simulink model "ASM_Traffic_MultiCore"  (R2026a)
settings: Solver=ode1  StartTime=SIM.tstart.v  StopTime=SIM.tend.v  FixedStep=SIM.StepSize.v
PostLoadFcn:
  | if any(exist('dsrtsu_mdlpostloadfcn', 'file') ~= 0), dsrtsu_mdlpostloadfcn('Execute', bdroot); end
  | try, asm_mdl_postloadfcn(bdroot, 'UpdateModel', 3600); catch, disp(lasterr); end,
InitFcn:
  | , if any(exist('rtifpga_mdlclblib', 'file') ~= 0), rtifpga_mdlclblib('Init', bdroot); end,
  | , if any(exist('dsmpb_private', 'file') ~= 0), dsmpb_private('dsmpb_mdlclblib', 'Init', bdroot); end,
model workspace (MAT data in the model file):
  asmReferencePath = [0 0.01 0.02 0.03 0.04 0.05 0.06 0.07 0.08 0.09 0.1 0.11 ... (350007 elements, 50001x7)]
  roadBounds : Simulink.Parameter (value not decoded)
  safetyAxes : Simulink.Parameter (value not decoded)
undefined symbols (not defined in the file): _to_, a0b2, ASM_BrakeHydraulics_DemoSystems, ASM_VehicleDynamics_DemoSystems, b98103fe8ad365046cd0, BrakeCircuit, controllerConfig, CPT, Crankshaft, DiscIntNeverNeededParam, dsmsi, FinalDriveAssembly, MDL, ModeSignals, mu, Pos_BrakePedal_Maneuver, rad, RefSignals, roadFamilyData, roadFamilyId, s_to_rpm, SIM, SoftECU, Suspension, Tire, Transmission
libraries: ASM_Traffic_lib x135, simulink x98, ASM_Utils_lib x77, ASM_VehicleDynamics_lib x70, ASM_Environment_lib x22, dsmpblib x20, dsmsilib x15, MDLD_Utils_lib x10, ASM_BrakeHydraulics_lib x3, sl_discontinuities x2
(part 60 of 65)

== system ASM_Traffic_MultiCore/Environment/Sensors/UserInterface/DISP_Plant/Object_Sensor_2D/Object_Sensor_2D_VisualizationData/Sensor_1_Front_Long ==
  Sensor : Inport
  Angle_Hor_Rel[deg] : Gain
  Angle_ScopeZone_Horizontal[deg] : Gain
  Angle_z_Orientation_Sensor_CoorSys_V[deg] : Gain
  Bus Selector : BusSelector  OutputSignals=Parameters.Sensor_Enable[0Off|1On],Parameters.Sensor_Detection_Mode[1Ray|2Sector],Parameters.Length_ScopeZone[m],Parameters.Pos_Sensor_Apex_CoorSys_V[x;y;z][m],Parameters.Angle_z_Orientation_Sensor_CoorSys_V[deg],Parameters.Angle_ScopeZone_Horizontal[deg],Parameters.SensorIdx[],SensorOutput.Object_ID[],SensorOutput.Distance[m],SensorOutput.Angle_Hor_Rel[deg]
  Distance[m] : Gain
  Length_ScopeZone[m] : Gain
  Object_ID[] : Gain
  Pos_Sensor_Apex_CoorSys_V[x;y;z][m] : Gain
  SensorIdx[] : Gain
  Sensor_Detection_Mode[1Ray|2Sector] : Gain
  Sensor_Enable[0Off|1On] : Gain
  Terminator{,1..9} (10 alike) : Terminator
  wires:
  Sensor/1 -> Bus Selector/1
  Bus Selector/1 -> Sensor_Enable[0Off|1On]/1  "<Sensor_Enable[0Off|1On]>"
  Sensor_Enable[0Off|1On]/1 -> Terminator/1
  Sensor_Detection_Mode[1Ray|2Sector]/1 -> Terminator1/1
  Bus Selector/2 -> Sensor_Detection_Mode[1Ray|2Sector]/1  "<Sensor_Detection_Mode[1Ray|2Sector]>"
  Pos_Sensor_Apex_CoorSys_V[x;y;z][m]/1 -> Terminator2/1
  Angle_z_Orientation_Sensor_CoorSys_V[deg]/1 -> Terminator3/1
  Angle_ScopeZone_Horizontal[deg]/1 -> Terminator4/1
  SensorIdx[]/1 -> Terminator5/1
  Object_ID[]/1 -> Terminator6/1
  Distance[m]/1 -> Terminator7/1
  Angle_Hor_Rel[deg]/1 -> Terminator8/1
  Bus Selector/4 -> Pos_Sensor_Apex_CoorSys_V[x;y;z][m]/1  "<Pos_Sensor_Apex_CoorSys_V[x;y;z][m]>"
  Bus Selector/5 -> Angle_z_Orientation_Sensor_CoorSys_V[deg]/1  "<Angle_z_Orientation_Sensor_CoorSys_V[deg]>"
  Bus Selector/6 -> Angle_ScopeZone_Horizontal[deg]/1  "<Angle_ScopeZone_Horizontal[deg]>"
  Bus Selector/7 -> SensorIdx[]/1  "<SensorIdx[]>"
  Bus Selector/8 -> Object_ID[]/1  "<Object_ID[]>"
  Bus Selector/9 -> Distance[m]/1  "<Distance[m]>"
  Bus Selector/10 -> Angle_Hor_Rel[deg]/1  "<Angle_Hor_Rel[deg]>"
  Length_ScopeZone[m]/1 -> Terminator9/1
  Bus Selector/3 -> Length_ScopeZone[m]/1  "<Length_ScopeZone[m]>"

== system ASM_Traffic_MultiCore/Environment/Sensors/UserInterface/DISP_Plant/Object_Sensor_2D/Object_Sensor_2D_VisualizationData/Sensor_2_Front_Left ==
  Sensor : Inport
  Angle_Hor_Rel[deg] : Gain
  Angle_ScopeZone_Horizontal[deg] : Gain
  Angle_z_Orientation_Sensor_CoorSys_V[deg] : Gain
  Bus Selector : BusSelector  OutputSignals=Parameters.Sensor_Enable[0Off|1On],Parameters.Sensor_Detection_Mode[1Ray|2Sector],Parameters.Length_ScopeZone[m],Parameters.Pos_Sensor_Apex_CoorSys_V[x;y;z][m],Parameters.Angle_z_Orientation_Sensor_CoorSys_V[deg],Parameters.Angle_ScopeZone_Horizontal[deg],Parameters.SensorIdx[],SensorOutput.Object_ID[],SensorOutput.Distance[m],SensorOutput.Angle_Hor_Rel[deg]
  Distance[m] : Gain
  Length_ScopeZone[m] : Gain
  Object_ID[] : Gain
  Pos_Sensor_Apex_CoorSys_V[x;y;z][m] : Gain
  SensorIdx[] : Gain
  Sensor_Detection_Mode[1Ray|2Sector] : Gain
  Sensor_Enable[0Off|1On] : Gain
  Terminator{,1..9} (10 alike) : Terminator
  wires:
  Bus Selector/3 -> Length_ScopeZone[m]/1  "<Length_ScopeZone[m]>"
  Length_ScopeZone[m]/1 -> Terminator9/1
  Bus Selector/10 -> Angle_Hor_Rel[deg]/1  "<Angle_Hor_Rel[deg]>"
  Bus Selector/9 -> Distance[m]/1  "<Distance[m]>"
  Bus Selector/8 -> Object_ID[]/1  "<Object_ID[]>"
  Bus Selector/7 -> SensorIdx[]/1  "<SensorIdx[]>"
  Bus Selector/6 -> Angle_ScopeZone_Horizontal[deg]/1  "<Angle_ScopeZone_Horizontal[deg]>"
  Bus Selector/5 -> Angle_z_Orientation_Sensor_CoorSys_V[deg]/1  "<Angle_z_Orientation_Sensor_CoorSys_V[deg]>"
  Bus Selector/4 -> Pos_Sensor_Apex_CoorSys_V[x;y;z][m]/1  "<Pos_Sensor_Apex_CoorSys_V[x;y;z][m]>"
  Angle_Hor_Rel[deg]/1 -> Terminator8/1
  Distance[m]/1 -> Terminator7/1
  Object_ID[]/1 -> Terminator6/1
  SensorIdx[]/1 -> Terminator5/1
  Angle_ScopeZone_Horizontal[deg]/1 -> Terminator4/1
  Angle_z_Orientation_Sensor_CoorSys_V[deg]/1 -> Terminator3/1
  Pos_Sensor_Apex_CoorSys_V[x;y;z][m]/1 -> Terminator2/1
  Bus Selector/2 -> Sensor_Detection_Mode[1Ray|2Sector]/1  "<Sensor_Detection_Mode[1Ray|2Sector]>"
  Sensor_Detection_Mode[1Ray|2Sector]/1 -> Terminator1/1
  Sensor_Enable[0Off|1On]/1 -> Terminator/1
  Bus Selector/1 -> Sensor_Enable[0Off|1On]/1  "<Sensor_Enable[0Off|1On]>"
  Sensor/1 -> Bus Selector/1

== system ASM_Traffic_MultiCore/Environment/Sensors/UserInterface/DISP_Plant/Object_Sensor_2D/Object_Sensor_2D_VisualizationData/Sensor_3_Left ==
  Sensor : Inport
  Angle_Hor_Rel[deg] : Gain
  Angle_ScopeZone_Horizontal[deg] : Gain
  Angle_z_Orientation_Sensor_CoorSys_V[deg] : Gain
  Bus Selector : BusSelector  OutputSignals=Parameters.Sensor_Enable[0Off|1On],Parameters.Sensor_Detection_Mode[1Ray|2Sector],Parameters.Length_ScopeZone[m],Parameters.Pos_Sensor_Apex_CoorSys_V[x;y;z][m],Parameters.Angle_z_Orientation_Sensor_CoorSys_V[deg],Parameters.Angle_ScopeZone_Horizontal[deg],Parameters.SensorIdx[],SensorOutput.Object_ID[],SensorOutput.Distance[m],SensorOutput.Angle_Hor_Rel[deg]
  Distance[m] : Gain
  Length_ScopeZone[m] : Gain
  Object_ID[] : Gain
  Pos_Sensor_Apex_CoorSys_V[x;y;z][m] : Gain
  SensorIdx[] : Gain
  Sensor_Detection_Mode[1Ray|2Sector] : Gain
  Sensor_Enable[0Off|1On] : Gain
  Terminator{,1..9} (10 alike) : Terminator
  wires:
  Sensor/1 -> Bus Selector/1
  Bus Selector/1 -> Sensor_Enable[0Off|1On]/1  "<Sensor_Enable[0Off|1On]>"
  Sensor_Enable[0Off|1On]/1 -> Terminator/1
  Sensor_Detection_Mode[1Ray|2Sector]/1 -> Terminator1/1
  Bus Selector/2 -> Sensor_Detection_Mode[1Ray|2Sector]/1  "<Sensor_Detection_Mode[1Ray|2Sector]>"
  Pos_Sensor_Apex_CoorSys_V[x;y;z][m]/1 -> Terminator2/1
  Angle_z_Orientation_Sensor_CoorSys_V[deg]/1 -> Terminator3/1
  Angle_ScopeZone_Horizontal[deg]/1 -> Terminator4/1
  SensorIdx[]/1 -> Terminator5/1
  Object_ID[]/1 -> Terminator6/1
  Distance[m]/1 -> Terminator7/1
  Angle_Hor_Rel[deg]/1 -> Terminator8/1
  Bus Selector/4 -> Pos_Sensor_Apex_CoorSys_V[x;y;z][m]/1  "<Pos_Sensor_Apex_CoorSys_V[x;y;z][m]>"
  Bus Selector/5 -> Angle_z_Orientation_Sensor_CoorSys_V[deg]/1  "<Angle_z_Orientation_Sensor_CoorSys_V[deg]>"
  Bus Selector/6 -> Angle_ScopeZone_Horizontal[deg]/1  "<Angle_ScopeZone_Horizontal[deg]>"
  Bus Selector/7 -> SensorIdx[]/1  "<SensorIdx[]>"
  Bus Selector/8 -> Object_ID[]/1  "<Object_ID[]>"
  Bus Selector/9 -> Distance[m]/1  "<Distance[m]>"
  Bus Selector/10 -> Angle_Hor_Rel[deg]/1  "<Angle_Hor_Rel[deg]>"
  Length_ScopeZone[m]/1 -> Terminator9/1
  Bus Selector/3 -> Length_ScopeZone[m]/1  "<Length_ScopeZone[m]>"

== system ASM_Traffic_MultiCore/Environment/Sensors/UserInterface/DISP_Plant/Object_Sensor_2D/Object_Sensor_2D_VisualizationData/Sensor_4_Rear_Left ==
  Sensor : Inport
  Angle_Hor_Rel[deg] : Gain
  Angle_ScopeZone_Horizontal[deg] : Gain
  Angle_z_Orientation_Sensor_CoorSys_V[deg] : Gain
  Bus Selector : BusSelector  OutputSignals=Parameters.Sensor_Enable[0Off|1On],Parameters.Sensor_Detection_Mode[1Ray|2Sector],Parameters.Length_ScopeZone[m],Parameters.Pos_Sensor_Apex_CoorSys_V[x;y;z][m],Parameters.Angle_z_Orientation_Sensor_CoorSys_V[deg],Parameters.Angle_ScopeZone_Horizontal[deg],Parameters.SensorIdx[],SensorOutput.Object_ID[],SensorOutput.Distance[m],SensorOutput.Angle_Hor_Rel[deg]
  Distance[m] : Gain
  Length_ScopeZone[m] : Gain
  Object_ID[] : Gain
  Pos_Sensor_Apex_CoorSys_V[x;y;z][m] : Gain
  SensorIdx[] : Gain
  Sensor_Detection_Mode[1Ray|2Sector] : Gain
  Sensor_Enable[0Off|1On] : Gain
  Terminator{,1..9} (10 alike) : Terminator
  wires:
  Bus Selector/3 -> Length_ScopeZone[m]/1  "<Length_ScopeZone[m]>"
  Length_ScopeZone[m]/1 -> Terminator9/1
  Bus Selector/10 -> Angle_Hor_Rel[deg]/1  "<Angle_Hor_Rel[deg]>"
  Bus Selector/9 -> Distance[m]/1  "<Distance[m]>"
  Bus Selector/8 -> Object_ID[]/1  "<Object_ID[]>"
  Bus Selector/7 -> SensorIdx[]/1  "<SensorIdx[]>"
  Bus Selector/6 -> Angle_ScopeZone_Horizontal[deg]/1  "<Angle_ScopeZone_Horizontal[deg]>"
  Bus Selector/5 -> Angle_z_Orientation_Sensor_CoorSys_V[deg]/1  "<Angle_z_Orientation_Sensor_CoorSys_V[deg]>"
  Bus Selector/4 -> Pos_Sensor_Apex_CoorSys_V[x;y;z][m]/1  "<Pos_Sensor_Apex_CoorSys_V[x;y;z][m]>"
  Angle_Hor_Rel[deg]/1 -> Terminator8/1
  Distance[m]/1 -> Terminator7/1
  Object_ID[]/1 -> Terminator6/1
  SensorIdx[]/1 -> Terminator5/1
  Angle_ScopeZone_Horizontal[deg]/1 -> Terminator4/1
  Angle_z_Orientation_Sensor_CoorSys_V[deg]/1 -> Terminator3/1
  Pos_Sensor_Apex_CoorSys_V[x;y;z][m]/1 -> Terminator2/1
  Bus Selector/2 -> Sensor_Detection_Mode[1Ray|2Sector]/1  "<Sensor_Detection_Mode[1Ray|2Sector]>"
  Sensor_Detection_Mode[1Ray|2Sector]/1 -> Terminator1/1
  Sensor_Enable[0Off|1On]/1 -> Terminator/1
  Bus Selector/1 -> Sensor_Enable[0Off|1On]/1  "<Sensor_Enable[0Off|1On]>"
  Sensor/1 -> Bus Selector/1

== system ASM_Traffic_MultiCore/Environment/Sensors/UserInterface/DISP_Plant/Object_Sensor_2D/Object_Sensor_2D_VisualizationData/Sensor_5_Front_Right ==
  Sensor : Inport
  Angle_Hor_Rel[deg] : Gain
  Angle_ScopeZone_Horizontal[deg] : Gain
  Angle_z_Orientation_Sensor_CoorSys_V[deg] : Gain
  Bus Selector : BusSelector  OutputSignals=Parameters.Sensor_Enable[0Off|1On],Parameters.Sensor_Detection_Mode[1Ray|2Sector],Parameters.Length_ScopeZone[m],Parameters.Pos_Sensor_Apex_CoorSys_V[x;y;z][m],Parameters.Angle_z_Orientation_Sensor_CoorSys_V[deg],Parameters.Angle_ScopeZone_Horizontal[deg],Parameters.SensorIdx[],SensorOutput.Object_ID[],SensorOutput.Distance[m],SensorOutput.Angle_Hor_Rel[deg]
  Distance[m] : Gain
  Length_ScopeZone[m] : Gain
  Object_ID[] : Gain
  Pos_Sensor_Apex_CoorSys_V[x;y;z][m] : Gain
  SensorIdx[] : Gain
  Sensor_Detection_Mode[1Ray|2Sector] : Gain
  Sensor_Enable[0Off|1On] : Gain
  Terminator{,1..9} (10 alike) : Terminator
  wires:
  Sensor/1 -> Bus Selector/1
  Bus Selector/1 -> Sensor_Enable[0Off|1On]/1  "<Sensor_Enable[0Off|1On]>"
  Sensor_Enable[0Off|1On]/1 -> Terminator/1
  Sensor_Detection_Mode[1Ray|2Sector]/1 -> Terminator1/1
  Bus Selector/2 -> Sensor_Detection_Mode[1Ray|2Sector]/1  "<Sensor_Detection_Mode[1Ray|2Sector]>"
  Pos_Sensor_Apex_CoorSys_V[x;y;z][m]/1 -> Terminator2/1
  Angle_z_Orientation_Sensor_CoorSys_V[deg]/1 -> Terminator3/1
  Angle_ScopeZone_Horizontal[deg]/1 -> Terminator4/1
  SensorIdx[]/1 -> Terminator5/1
  Object_ID[]/1 -> Terminator6/1
  Distance[m]/1 -> Terminator7/1
  Angle_Hor_Rel[deg]/1 -> Terminator8/1
  Bus Selector/4 -> Pos_Sensor_Apex_CoorSys_V[x;y;z][m]/1  "<Pos_Sensor_Apex_CoorSys_V[x;y;z][m]>"
  Bus Selector/5 -> Angle_z_Orientation_Sensor_CoorSys_V[deg]/1  "<Angle_z_Orientation_Sensor_CoorSys_V[deg]>"
  Bus Selector/6 -> Angle_ScopeZone_Horizontal[deg]/1  "<Angle_ScopeZone_Horizontal[deg]>"
  Bus Selector/7 -> SensorIdx[]/1  "<SensorIdx[]>"
  Bus Selector/8 -> Object_ID[]/1  "<Object_ID[]>"
  Bus Selector/9 -> Distance[m]/1  "<Distance[m]>"
  Bus Selector/10 -> Angle_Hor_Rel[deg]/1  "<Angle_Hor_Rel[deg]>"
  Length_ScopeZone[m]/1 -> Terminator9/1
  Bus Selector/3 -> Length_ScopeZone[m]/1  "<Length_ScopeZone[m]>"

== system ASM_Traffic_MultiCore/Environment/Sensors/UserInterface/DISP_Plant/Object_Sensor_2D/Object_Sensor_2D_VisualizationData/Sensor_6_Right ==
  Sensor : Inport
  Angle_Hor_Rel[deg] : Gain
  Angle_ScopeZone_Horizontal[deg] : Gain
  Angle_z_Orientation_Sensor_CoorSys_V[deg] : Gain
  Bus Selector : BusSelector  OutputSignals=Parameters.Sensor_Enable[0Off|1On],Parameters.Sensor_Detection_Mode[1Ray|2Sector],Parameters.Length_ScopeZone[m],Parameters.Pos_Sensor_Apex_CoorSys_V[x;y;z][m],Parameters.Angle_z_Orientation_Sensor_CoorSys_V[deg],Parameters.Angle_ScopeZone_Horizontal[deg],Parameters.SensorIdx[],SensorOutput.Object_ID[],SensorOutput.Distance[m],SensorOutput.Angle_Hor_Rel[deg]
  Distance[m] : Gain
  Length_ScopeZone[m] : Gain
  Object_ID[] : Gain
  Pos_Sensor_Apex_CoorSys_V[x;y;z][m] : Gain
  SensorIdx[] : Gain
  Sensor_Detection_Mode[1Ray|2Sector] : Gain
  Sensor_Enable[0Off|1On] : Gain
  Terminator{,1..9} (10 alike) : Terminator
  wires:
  Bus Selector/3 -> Length_ScopeZone[m]/1  "<Length_ScopeZone[m]>"
  Length_ScopeZone[m]/1 -> Terminator9/1
  Bus Selector/10 -> Angle_Hor_Rel[deg]/1  "<Angle_Hor_Rel[deg]>"
  Bus Selector/9 -> Distance[m]/1  "<Distance[m]>"
  Bus Selector/8 -> Object_ID[]/1  "<Object_ID[]>"
  Bus Selector/7 -> SensorIdx[]/1  "<SensorIdx[]>"
  Bus Selector/6 -> Angle_ScopeZone_Horizontal[deg]/1  "<Angle_ScopeZone_Horizontal[deg]>"
  Bus Selector/5 -> Angle_z_Orientation_Sensor_CoorSys_V[deg]/1  "<Angle_z_Orientation_Sensor_CoorSys_V[deg]>"
  Bus Selector/4 -> Pos_Sensor_Apex_CoorSys_V[x;y;z][m]/1  "<Pos_Sensor_Apex_CoorSys_V[x;y;z][m]>"
  Angle_Hor_Rel[deg]/1 -> Terminator8/1
  Distance[m]/1 -> Terminator7/1
  Object_ID[]/1 -> Terminator6/1
  SensorIdx[]/1 -> Terminator5/1
  Angle_ScopeZone_Horizontal[deg]/1 -> Terminator4/1
  Angle_z_Orientation_Sensor_CoorSys_V[deg]/1 -> Terminator3/1
  Pos_Sensor_Apex_CoorSys_V[x;y;z][m]/1 -> Terminator2/1
  Bus Selector/2 -> Sensor_Detection_Mode[1Ray|2Sector]/1  "<Sensor_Detection_Mode[1Ray|2Sector]>"
  Sensor_Detection_Mode[1Ray|2Sector]/1 -> Terminator1/1
  Sensor_Enable[0Off|1On]/1 -> Terminator/1
  Bus Selector/1 -> Sensor_Enable[0Off|1On]/1  "<Sensor_Enable[0Off|1On]>"
  Sensor/1 -> Bus Selector/1

== system ASM_Traffic_MultiCore/Environment/Sensors/UserInterface/DISP_Plant/Object_Sensor_2D/Object_Sensor_2D_VisualizationData/Sensor_7_Rear_Right ==
  Sensor : Inport
  Angle_Hor_Rel[deg] : Gain
  Angle_ScopeZone_Horizontal[deg] : Gain
  Angle_z_Orientation_Sensor_CoorSys_V[deg] : Gain
  Bus Selector : BusSelector  OutputSignals=Parameters.Sensor_Enable[0Off|1On],Parameters.Sensor_Detection_Mode[1Ray|2Sector],Parameters.Length_ScopeZone[m],Parameters.Pos_Sensor_Apex_CoorSys_V[x;y;z][m],Parameters.Angle_z_Orientation_Sensor_CoorSys_V[deg],Parameters.Angle_ScopeZone_Horizontal[deg],Parameters.SensorIdx[],SensorOutput.Object_ID[],SensorOutput.Distance[m],SensorOutput.Angle_Hor_Rel[deg]
  Distance[m] : Gain
  Length_ScopeZone[m] : Gain
  Object_ID[] : Gain
  Pos_Sensor_Apex_CoorSys_V[x;y;z][m] : Gain
  SensorIdx[] : Gain
  Sensor_Detection_Mode[1Ray|2Sector] : Gain
  Sensor_Enable[0Off|1On] : Gain
  Terminator{,1..9} (10 alike) : Terminator
  wires:
  Sensor/1 -> Bus Selector/1
  Bus Selector/1 -> Sensor_Enable[0Off|1On]/1  "<Sensor_Enable[0Off|1On]>"
  Sensor_Enable[0Off|1On]/1 -> Terminator/1
  Sensor_Detection_Mode[1Ray|2Sector]/1 -> Terminator1/1
  Bus Selector/2 -> Sensor_Detection_Mode[1Ray|2Sector]/1  "<Sensor_Detection_Mode[1Ray|2Sector]>"
  Pos_Sensor_Apex_CoorSys_V[x;y;z][m]/1 -> Terminator2/1
  Angle_z_Orientation_Sensor_CoorSys_V[deg]/1 -> Terminator3/1
  Angle_ScopeZone_Horizontal[deg]/1 -> Terminator4/1
  SensorIdx[]/1 -> Terminator5/1
  Object_ID[]/1 -> Terminator6/1
  Distance[m]/1 -> Terminator7/1
  Angle_Hor_Rel[deg]/1 -> Terminator8/1
  Bus Selector/4 -> Pos_Sensor_Apex_CoorSys_V[x;y;z][m]/1  "<Pos_Sensor_Apex_CoorSys_V[x;y;z][m]>"
  Bus Selector/5 -> Angle_z_Orientation_Sensor_CoorSys_V[deg]/1  "<Angle_z_Orientation_Sensor_CoorSys_V[deg]>"
  Bus Selector/6 -> Angle_ScopeZone_Horizontal[deg]/1  "<Angle_ScopeZone_Horizontal[deg]>"
  Bus Selector/7 -> SensorIdx[]/1  "<SensorIdx[]>"
  Bus Selector/8 -> Object_ID[]/1  "<Object_ID[]>"
  Bus Selector/9 -> Distance[m]/1  "<Distance[m]>"
  Bus Selector/10 -> Angle_Hor_Rel[deg]/1  "<Angle_Hor_Rel[deg]>"
  Length_ScopeZone[m]/1 -> Terminator9/1
  Bus Selector/3 -> Length_ScopeZone[m]/1  "<Length_ScopeZone[m]>"

== system ASM_Traffic_MultiCore/Environment/Sensors/UserInterface/DISP_Plant/Object_Sensor_3D/IdxSelect_3DSensor/Angle_Hor_Object_1[deg] ==
  In1 : Inport
  Out1 : Outport  VectorParamsAs1DForOutWhenUnconnected=off
  wires:
  In1/1 -> Out1/1

== system ASM_Traffic_MultiCore/Environment/Sensors/UserInterface/DISP_Plant/Object_Sensor_3D/IdxSelect_3DSensor/Angle_Hor_Object_2[deg] ==
  In1 : Inport
  Out1 : Outport  VectorParamsAs1DForOutWhenUnconnected=off
  wires:
  In1/1 -> Out1/1

== system ASM_Traffic_MultiCore/Environment/Sensors/UserInterface/DISP_Plant/Object_Sensor_3D/IdxSelect_3DSensor/Angle_Hor_Object_3[deg] ==
  In1 : Inport
  Out1 : Outport  VectorParamsAs1DForOutWhenUnconnected=off
  wires:
  In1/1 -> Out1/1

== system ASM_Traffic_MultiCore/Environment/Sensors/UserInterface/DISP_Plant/Object_Sensor_3D/IdxSelect_3DSensor/Angle_Ver_Object_1[deg] ==
  In1 : Inport
  Out1 : Outport  VectorParamsAs1DForOutWhenUnconnected=off
  wires:
  In1/1 -> Out1/1

== system ASM_Traffic_MultiCore/Environment/Sensors/UserInterface/DISP_Plant/Object_Sensor_3D/IdxSelect_3DSensor/Angle_Ver_Object_2[deg] ==
  In1 : Inport
  Out1 : Outport  VectorParamsAs1DForOutWhenUnconnected=off
  wires:
  In1/1 -> Out1/1

== system ASM_Traffic_MultiCore/Environment/Sensors/UserInterface/DISP_Plant/Object_Sensor_3D/IdxSelect_3DSensor/Angle_Ver_Object_3[deg] ==
  In1 : Inport
  Out1 : Outport  VectorParamsAs1DForOutWhenUnconnected=off
  wires:
  In1/1 -> Out1/1

== system ASM_Traffic_MultiCore/Environment/Sensors/UserInterface/DISP_Plant/Object_Sensor_3D/IdxSelect_3DSensor/Angle_x_Objects_CoorSysE_1[deg] ==
  In1 : Inport
  Out1 : Outport  VectorParamsAs1DForOutWhenUnconnected=off
  wires:
  In1/1 -> Out1/1

== system ASM_Traffic_MultiCore/Environment/Sensors/UserInterface/DISP_Plant/Object_Sensor_3D/IdxSelect_3DSensor/Angle_x_Objects_CoorSysE_2[deg] ==
  In1 : Inport
  Out1 : Outport  VectorParamsAs1DForOutWhenUnconnected=off
  wires:
  In1/1 -> Out1/1

== system ASM_Traffic_MultiCore/Environment/Sensors/UserInterface/DISP_Plant/Object_Sensor_3D/IdxSelect_3DSensor/Angle_x_Objects_CoorSysE_3[deg] ==
  In1 : Inport
  Out1 : Outport  VectorParamsAs1DForOutWhenUnconnected=off
  wires:
  In1/1 -> Out1/1

== system ASM_Traffic_MultiCore/Environment/Sensors/UserInterface/DISP_Plant/Object_Sensor_3D/IdxSelect_3DSensor/Angle_y_Objects_CoorSysE_1[deg] ==
  In1 : Inport
  Out1 : Outport  VectorParamsAs1DForOutWhenUnconnected=off
  wires:
  In1/1 -> Out1/1

== system ASM_Traffic_MultiCore/Environment/Sensors/UserInterface/DISP_Plant/Object_Sensor_3D/IdxSelect_3DSensor/Angle_y_Objects_CoorSysE_2[deg] ==
  In1 : Inport
  Out1 : Outport  VectorParamsAs1DForOutWhenUnconnected=off
  wires:
  In1/1 -> Out1/1

== system ASM_Traffic_MultiCore/Environment/Sensors/UserInterface/DISP_Plant/Object_Sensor_3D/IdxSelect_3DSensor/Angle_y_Objects_CoorSysE_3[deg] ==
  In1 : Inport
  Out1 : Outport  VectorParamsAs1DForOutWhenUnconnected=off
  wires:
  In1/1 -> Out1/1

== system ASM_Traffic_MultiCore/Environment/Sensors/UserInterface/DISP_Plant/Object_Sensor_3D/IdxSelect_3DSensor/Angle_z_Objects_CoorSysE_1[deg] ==
  In1 : Inport
  Out1 : Outport  VectorParamsAs1DForOutWhenUnconnected=off
  wires:
  In1/1 -> Out1/1

== system ASM_Traffic_MultiCore/Environment/Sensors/UserInterface/DISP_Plant/Object_Sensor_3D/IdxSelect_3DSensor/Angle_z_Objects_CoorSysE_2[deg] ==
  In1 : Inport
  Out1 : Outport  VectorParamsAs1DForOutWhenUnconnected=off
  wires:
  In1/1 -> Out1/1

== system ASM_Traffic_MultiCore/Environment/Sensors/UserInterface/DISP_Plant/Object_Sensor_3D/IdxSelect_3DSensor/Angle_z_Objects_CoorSysE_3[deg] ==
  In1 : Inport
  Out1 : Outport  VectorParamsAs1DForOutWhenUnconnected=off
  wires:
  In1/1 -> Out1/1

== system ASM_Traffic_MultiCore/Environment/Sensors/UserInterface/DISP_Plant/Object_Sensor_3D/IdxSelect_3DSensor/CustomPoint_Angle_Hor_CoorSys_S_1[deg] ==
  In1 : Inport
  Out1 : Outport  VectorParamsAs1DForOutWhenUnconnected=off
  wires:
  In1/1 -> Out1/1

== system ASM_Traffic_MultiCore/Environment/Sensors/UserInterface/DISP_Plant/Object_Sensor_3D/IdxSelect_3DSensor/CustomPoint_Angle_Hor_CoorSys_S_2[deg] ==
  In1 : Inport
  Out1 : Outport  VectorParamsAs1DForOutWhenUnconnected=off
  wires:
  In1/1 -> Out1/1

== system ASM_Traffic_MultiCore/Environment/Sensors/UserInterface/DISP_Plant/Object_Sensor_3D/IdxSelect_3DSensor/CustomPoint_Angle_Hor_CoorSys_S_3[deg] ==
  In1 : Inport
  Out1 : Outport  VectorParamsAs1DForOutWhenUnconnected=off
  wires:
  In1/1 -> Out1/1

== system ASM_Traffic_MultiCore/Environment/Sensors/UserInterface/DISP_Plant/Object_Sensor_3D/IdxSelect_3DSensor/CustomPoint_Dist_CoorSys_S_1[m] ==
  In1 : Inport
  Out1 : Outport  VectorParamsAs1DForOutWhenUnconnected=off
  wires:
  In1/1 -> Out1/1

== system ASM_Traffic_MultiCore/Environment/Sensors/UserInterface/DISP_Plant/Object_Sensor_3D/IdxSelect_3DSensor/CustomPoint_Dist_CoorSys_S_2[m] ==
  In1 : Inport
  Out1 : Outport  VectorParamsAs1DForOutWhenUnconnected=off
  wires:
  In1/1 -> Out1/1

== system ASM_Traffic_MultiCore/Environment/Sensors/UserInterface/DISP_Plant/Object_Sensor_3D/IdxSelect_3DSensor/CustomPoint_Dist_CoorSys_S_3[m] ==
  In1 : Inport
  Out1 : Outport  VectorParamsAs1DForOutWhenUnconnected=off
  wires:
  In1/1 -> Out1/1

== system ASM_Traffic_MultiCore/Environment/Sensors/UserInterface/DISP_Plant/Object_Sensor_3D/IdxSelect_3DSensor/CustomPoint_ID_1[] ==
  In1 : Inport
  Out1 : Outport  VectorParamsAs1DForOutWhenUnconnected=off
  wires:
  In1/1 -> Out1/1

== system ASM_Traffic_MultiCore/Environment/Sensors/UserInterface/DISP_Plant/Object_Sensor_3D/IdxSelect_3DSensor/CustomPoint_ID_2[] ==
  In1 : Inport
  Out1 : Outport  VectorParamsAs1DForOutWhenUnconnected=off
  wires:
  In1/1 -> Out1/1

== system ASM_Traffic_MultiCore/Environment/Sensors/UserInterface/DISP_Plant/Object_Sensor_3D/IdxSelect_3DSensor/CustomPoint_ID_3[] ==
  In1 : Inport
  Out1 : Outport  VectorParamsAs1DForOutWhenUnconnected=off
  wires:
  In1/1 -> Out1/1

== system ASM_Traffic_MultiCore/Environment/Sensors/UserInterface/DISP_Plant/Object_Sensor_3D/IdxSelect_3DSensor/CustomPoint_Pos_ObjectPoint_CoorSys_E_1[x;y;z][m] ==
  In1 : Inport
  Out1 : Outport  VectorParamsAs1DForOutWhenUnconnected=off
  wires:
  In1/1 -> Out1/1

== system ASM_Traffic_MultiCore/Environment/Sensors/UserInterface/DISP_Plant/Object_Sensor_3D/IdxSelect_3DSensor/CustomPoint_Pos_ObjectPoint_CoorSys_E_2[x;y;z][m] ==
  In1 : Inport
  Out1 : Outport  VectorParamsAs1DForOutWhenUnconnected=off
  wires:
  In1/1 -> Out1/1

== system ASM_Traffic_MultiCore/Environment/Sensors/UserInterface/DISP_Plant/Object_Sensor_3D/IdxSelect_3DSensor/CustomPoint_Pos_ObjectPoint_CoorSys_E_3[x;y;z][m] ==
  In1 : Inport
  Out1 : Outport  VectorParamsAs1DForOutWhenUnconnected=off
  wires:
  In1/1 -> Out1/1

== system ASM_Traffic_MultiCore/Environment/Sensors/UserInterface/DISP_Plant/Object_Sensor_3D/IdxSelect_3DSensor/CustomValues_1[] ==
  In1 : Inport
  Out1 : Outport  VectorParamsAs1DForOutWhenUnconnected=off
  wires:
  In1/1 -> Out1/1

== system ASM_Traffic_MultiCore/Environment/Sensors/UserInterface/DISP_Plant/Object_Sensor_3D/IdxSelect_3DSensor/CustomValues_2[] ==
  In1 : Inport
  Out1 : Outport  VectorParamsAs1DForOutWhenUnconnected=off
  wires:
  In1/1 -> Out1/1

== system ASM_Traffic_MultiCore/Environment/Sensors/UserInterface/DISP_Plant/Object_Sensor_3D/IdxSelect_3DSensor/CustomValues_3[] ==
  In1 : Inport
  Out1 : Outport  VectorParamsAs1DForOutWhenUnconnected=off
  wires:
  In1/1 -> Out1/1

== system ASM_Traffic_MultiCore/Environment/Sensors/UserInterface/DISP_Plant/Object_Sensor_3D/IdxSelect_3DSensor/Dist_Object_1[m] ==
  In1 : Inport
  Out1 : Outport  VectorParamsAs1DForOutWhenUnconnected=off
  wires:
  In1/1 -> Out1/1

== system ASM_Traffic_MultiCore/Environment/Sensors/UserInterface/DISP_Plant/Object_Sensor_3D/IdxSelect_3DSensor/Dist_Object_2[m] ==
  In1 : Inport
  Out1 : Outport  VectorParamsAs1DForOutWhenUnconnected=off
  wires:
  In1/1 -> Out1/1

== system ASM_Traffic_MultiCore/Environment/Sensors/UserInterface/DISP_Plant/Object_Sensor_3D/IdxSelect_3DSensor/Dist_Object_3[m] ==
  In1 : Inport
  Out1 : Outport  VectorParamsAs1DForOutWhenUnconnected=off
  wires:
  In1/1 -> Out1/1

== system ASM_Traffic_MultiCore/Environment/Sensors/UserInterface/DISP_Plant/Object_Sensor_3D/IdxSelect_3DSensor/Flag_BoxProperties_1[0|1] ==
  In1 : Inport
  Out1 : Outport  VectorParamsAs1DForOutWhenUnconnected=off
  wires:
  In1/1 -> Out1/1

== system ASM_Traffic_MultiCore/Environment/Sensors/UserInterface/DISP_Plant/Object_Sensor_3D/IdxSelect_3DSensor/Flag_BoxProperties_2[0|1] ==
  In1 : Inport
  Out1 : Outport  VectorParamsAs1DForOutWhenUnconnected=off
  wires:
  In1/1 -> Out1/1

== system ASM_Traffic_MultiCore/Environment/Sensors/UserInterface/DISP_Plant/Object_Sensor_3D/IdxSelect_3DSensor/Flag_BoxProperties_3[0|1] ==
  In1 : Inport
  Out1 : Outport  VectorParamsAs1DForOutWhenUnconnected=off
  wires:
  In1/1 -> Out1/1

== system ASM_Traffic_MultiCore/Environment/Sensors/UserInterface/DISP_Plant/Object_Sensor_3D/IdxSelect_3DSensor/Flag_NearestPnt_Occluded1[-1|0|1] ==
  In1 : Inport
  Out1 : Outport  VectorParamsAs1DForOutWhenUnconnected=off
  wires:
  In1/1 -> Out1/1

== system ASM_Traffic_MultiCore/Environment/Sensors/UserInterface/DISP_Plant/Object_Sensor_3D/IdxSelect_3DSensor/Flag_NearestPnt_Occluded2[-1|0|1] ==
  In1 : Inport
  Out1 : Outport  VectorParamsAs1DForOutWhenUnconnected=off
  wires:
  In1/1 -> Out1/1

== system ASM_Traffic_MultiCore/Environment/Sensors/UserInterface/DISP_Plant/Object_Sensor_3D/IdxSelect_3DSensor/Flag_NearestPnt_Occluded3[-1|0|1] ==
  In1 : Inport
  Out1 : Outport  VectorParamsAs1DForOutWhenUnconnected=off
  wires:
  In1/1 -> Out1/1

== system ASM_Traffic_MultiCore/Environment/Sensors/UserInterface/DISP_Plant/Object_Sensor_3D/IdxSelect_3DSensor/Flag_Object_In_Scope_1[0Out|1In] ==
  In1 : Inport
  Out1 : Outport  VectorParamsAs1DForOutWhenUnconnected=off
  wires:
  In1/1 -> Out1/1

== system ASM_Traffic_MultiCore/Environment/Sensors/UserInterface/DISP_Plant/Object_Sensor_3D/IdxSelect_3DSensor/Flag_Object_In_Scope_2[0Out|1In] ==
  In1 : Inport
  Out1 : Outport  VectorParamsAs1DForOutWhenUnconnected=off
  wires:
  In1/1 -> Out1/1

== system ASM_Traffic_MultiCore/Environment/Sensors/UserInterface/DISP_Plant/Object_Sensor_3D/IdxSelect_3DSensor/Flag_Object_In_Scope_3[0Out|1In] ==
  In1 : Inport
  Out1 : Outport  VectorParamsAs1DForOutWhenUnconnected=off
  wires:
  In1/1 -> Out1/1

== system ASM_Traffic_MultiCore/Environment/Sensors/UserInterface/DISP_Plant/Object_Sensor_3D/IdxSelect_3DSensor/Flag_Sensor_Apex_In_Object_1[0Out|1In] ==
  In1 : Inport
  Out1 : Outport  VectorParamsAs1DForOutWhenUnconnected=off
  wires:
  In1/1 -> Out1/1

== system ASM_Traffic_MultiCore/Environment/Sensors/UserInterface/DISP_Plant/Object_Sensor_3D/IdxSelect_3DSensor/Flag_Sensor_Apex_In_Object_2[0Out|1In] ==
  In1 : Inport
  Out1 : Outport  VectorParamsAs1DForOutWhenUnconnected=off
  wires:
  In1/1 -> Out1/1

== system ASM_Traffic_MultiCore/Environment/Sensors/UserInterface/DISP_Plant/Object_Sensor_3D/IdxSelect_3DSensor/Flag_Sensor_Apex_In_Object_3[0Out|1In] ==
  In1 : Inport
  Out1 : Outport  VectorParamsAs1DForOutWhenUnconnected=off
  wires:
  In1/1 -> Out1/1

== system ASM_Traffic_MultiCore/Environment/Sensors/UserInterface/DISP_Plant/Object_Sensor_3D/IdxSelect_3DSensor/Height_Object_1[m] ==
  In1 : Inport
  Out1 : Outport  VectorParamsAs1DForOutWhenUnconnected=off
  wires:
  In1/1 -> Out1/1

== system ASM_Traffic_MultiCore/Environment/Sensors/UserInterface/DISP_Plant/Object_Sensor_3D/IdxSelect_3DSensor/Height_Object_2[m] ==
  In1 : Inport
  Out1 : Outport  VectorParamsAs1DForOutWhenUnconnected=off
  wires:
  In1/1 -> Out1/1

== system ASM_Traffic_MultiCore/Environment/Sensors/UserInterface/DISP_Plant/Object_Sensor_3D/IdxSelect_3DSensor/Height_Object_3[m] ==
  In1 : Inport
  Out1 : Outport  VectorParamsAs1DForOutWhenUnconnected=off
  wires:
  In1/1 -> Out1/1

== system ASM_Traffic_MultiCore/Environment/Sensors/UserInterface/DISP_Plant/Object_Sensor_3D/IdxSelect_3DSensor/Length_Object_1[m] ==
  In1 : Inport
  Out1 : Outport  VectorParamsAs1DForOutWhenUnconnected=off
  wires:
  In1/1 -> Out1/1

== system ASM_Traffic_MultiCore/Environment/Sensors/UserInterface/DISP_Plant/Object_Sensor_3D/IdxSelect_3DSensor/Length_Object_2[m] ==
  In1 : Inport
  Out1 : Outport  VectorParamsAs1DForOutWhenUnconnected=off
  wires:
  In1/1 -> Out1/1

== system ASM_Traffic_MultiCore/Environment/Sensors/UserInterface/DISP_Plant/Object_Sensor_3D/IdxSelect_3DSensor/Length_Object_3[m] ==
  In1 : Inport
  Out1 : Outport  VectorParamsAs1DForOutWhenUnconnected=off
  wires:
  In1/1 -> Out1/1

== system ASM_Traffic_MultiCore/Environment/Sensors/UserInterface/DISP_Plant/Object_Sensor_3D/IdxSelect_3DSensor/MaskObjectData_CustomPoints_1 ==
  Object_ID_Expected[] : Inport
  Object_ID[] : Inport  Port=2
  ID[] : Inport  Port=3
  Dist_CoorSys_S[m] : Inport  Port=4
  Angle_Hor_CoorSys_S[deg] : Inport  Port=5
  Pos_ObjectPoint_CoorSys_E[x;y;z][m] : Inport  Port=6
  Demux : Demux  Outputs=3
  Mux : Mux  Inputs=3
  Product{,1..6} (7 alike) : Product
  Relational Operator1 : RelationalOperator  Operator===  OutDataTypeStr=boolean  RndMeth=Simplest  InputSameDT=off
  Object_ID_Masked[] : Outport
  ID_Masked[] : Outport  Port=2
  Dist_CoorSys_S_Masked[m] : Outport  Port=3
  Angle_Hor_CoorSys_S_Masked[deg] : Outport  Port=4
  Pos_ObjectPoint_CoorSys_E_Masked[x;y;z][m] : Outport  Port=5
  wires:
  Product6/1 -> Object_ID_Masked[]/1
  Demux/1 -> Product2/2
  Product5/1 -> Mux/3
  Product4/1 -> Mux/2
  Demux/2 -> Product4/2
  Relational Operator1/1 -> Product3/1, Product2/1, Product4/1, Product5/1, Product1/1, Product/1, Product6/1
  Product2/1 -> Mux/1
  Pos_ObjectPoint_CoorSys_E[x;y;z][m]/1 -> Demux/1
  Demux/3 -> Product5/2
  Object_ID[]/1 -> Relational Operator1/2, Product6/2
  Product1/1 -> Dist_CoorSys_S_Masked[m]/1
  Product3/1 -> Angle_Hor_CoorSys_S_Masked[deg]/1
  ID[]/1 -> Product/2
  Object_ID_Expected[]/1 -> Relational Operator1/1
  Product/1 -> ID_Masked[]/1
  Mux/1 -> Pos_ObjectPoint_CoorSys_E_Masked[x;y;z][m]/1
  Angle_Hor_CoorSys_S[deg]/1 -> Product3/2
  Dist_CoorSys_S[m]/1 -> Product1/2

== system ASM_Traffic_MultiCore/Environment/Sensors/UserInterface/DISP_Plant/Object_Sensor_3D/IdxSelect_3DSensor/MaskObjectData_CustomPoints_2 ==
  Object_ID_Expected[] : Inport
  Object_ID[] : Inport  Port=2
  ID[] : Inport  Port=3
  Dist_CoorSys_S[m] : Inport  Port=4
  Angle_Hor_CoorSys_S[deg] : Inport  Port=5
  Pos_ObjectPoint_CoorSys_E[x;y;z][m] : Inport  Port=6
  Demux : Demux  Outputs=3
  Mux : Mux  Inputs=3
  Product{,1..6} (7 alike) : Product
  Relational Operator1 : RelationalOperator  Operator===  OutDataTypeStr=boolean  RndMeth=Simplest  InputSameDT=off
  Object_ID_Masked[] : Outport
  ID_Masked[] : Outport  Port=2
  Dist_CoorSys_S_Masked[m] : Outport  Port=3
  Angle_Hor_CoorSys_S_Masked[deg] : Outport  Port=4
  Pos_ObjectPoint_CoorSys_E_Masked[x;y;z][m] : Outport  Port=5
  wires:
  Product6/1 -> Object_ID_Masked[]/1
  Demux/1 -> Product2/2
  Product5/1 -> Mux/3
  Product4/1 -> Mux/2
  Demux/2 -> Product4/2
  Relational Operator1/1 -> Product3/1, Product2/1, Product4/1, Product5/1, Product1/1, Product/1, Product6/1
  Product2/1 -> Mux/1
  Pos_ObjectPoint_CoorSys_E[x;y;z][m]/1 -> Demux/1
  Demux/3 -> Product5/2
  Object_ID[]/1 -> Relational Operator1/2, Product6/2
  Product1/1 -> Dist_CoorSys_S_Masked[m]/1
  Product3/1 -> Angle_Hor_CoorSys_S_Masked[deg]/1
  ID[]/1 -> Product/2
  Object_ID_Expected[]/1 -> Relational Operator1/1
  Product/1 -> ID_Masked[]/1
  Mux/1 -> Pos_ObjectPoint_CoorSys_E_Masked[x;y;z][m]/1
  Angle_Hor_CoorSys_S[deg]/1 -> Product3/2
  Dist_CoorSys_S[m]/1 -> Product1/2

== system ASM_Traffic_MultiCore/Environment/Sensors/UserInterface/DISP_Plant/Object_Sensor_3D/IdxSelect_3DSensor/MaskObjectData_CustomPoints_3 ==
  Object_ID_Expected[] : Inport
  Object_ID[] : Inport  Port=2
  ID[] : Inport  Port=3
  Dist_CoorSys_S[m] : Inport  Port=4
  Angle_Hor_CoorSys_S[deg] : Inport  Port=5
  Pos_ObjectPoint_CoorSys_E[x;y;z][m] : Inport  Port=6
  Demux : Demux  Outputs=3
  Mux : Mux  Inputs=3
  Product{,1..6} (7 alike) : Product
  Relational Operator1 : RelationalOperator  Operator===  OutDataTypeStr=boolean  RndMeth=Simplest  InputSameDT=off
  Object_ID_Masked[] : Outport
  ID_Masked[] : Outport  Port=2
  Dist_CoorSys_S_Masked[m] : Outport  Port=3
  Angle_Hor_CoorSys_S_Masked[deg] : Outport  Port=4
  Pos_ObjectPoint_CoorSys_E_Masked[x;y;z][m] : Outport  Port=5
  wires:
  Product6/1 -> Object_ID_Masked[]/1
  Demux/1 -> Product2/2
  Product5/1 -> Mux/3
  Product4/1 -> Mux/2
  Demux/2 -> Product4/2
  Relational Operator1/1 -> Product3/1, Product2/1, Product4/1, Product5/1, Product1/1, Product/1, Product6/1
  Product2/1 -> Mux/1
  Pos_ObjectPoint_CoorSys_E[x;y;z][m]/1 -> Demux/1
  Demux/3 -> Product5/2
  Object_ID[]/1 -> Relational Operator1/2, Product6/2
  Product1/1 -> Dist_CoorSys_S_Masked[m]/1
  Product3/1 -> Angle_Hor_CoorSys_S_Masked[deg]/1
  ID[]/1 -> Product/2
  Object_ID_Expected[]/1 -> Relational Operator1/1
  Product/1 -> ID_Masked[]/1
  Mux/1 -> Pos_ObjectPoint_CoorSys_E_Masked[x;y;z][m]/1
  Angle_Hor_CoorSys_S[deg]/1 -> Product3/2
  Dist_CoorSys_S[m]/1 -> Product1/2

== system ASM_Traffic_MultiCore/Environment/Sensors/UserInterface/DISP_Plant/Object_Sensor_3D/IdxSelect_3DSensor/MaskObjectData_RadarPoints_1 ==
  Object_ID_Expected[] : Inport
  Object_ID[] : Inport  Port=2
  ID[] : Inport  Port=3
  Dist_CoorSys_S[m] : Inport  Port=4
  Angle_Hor_CoorSys_S[deg] : Inport  Port=5
  Pos_ObjectPoint_CoorSys_E[x;y;z][m] : Inport  Port=6
  Demux : Demux  Outputs=3
  Mux : Mux  Inputs=3
  Product{,1..6} (7 alike) : Product
  Relational Operator1 : RelationalOperator  Operator===  OutDataTypeStr=boolean  RndMeth=Simplest  InputSameDT=off
  Object_ID_Masked[] : Outport
  ID_Masked[] : Outport  Port=2
  Dist_CoorSys_S_Masked[m] : Outport  Port=3
  Angle_Hor_CoorSys_S_Masked[deg] : Outport  Port=4
  Pos_ObjectPoint_CoorSys_E_Masked[x;y;z][m] : Outport  Port=5
  wires:
  Dist_CoorSys_S[m]/1 -> Product1/2
  Angle_Hor_CoorSys_S[deg]/1 -> Product3/2
  Mux/1 -> Pos_ObjectPoint_CoorSys_E_Masked[x;y;z][m]/1
  Product/1 -> ID_Masked[]/1
  Object_ID_Expected[]/1 -> Relational Operator1/1
  ID[]/1 -> Product/2
  Product3/1 -> Angle_Hor_CoorSys_S_Masked[deg]/1
  Product1/1 -> Dist_CoorSys_S_Masked[m]/1
  Object_ID[]/1 -> Product6/2, Relational Operator1/2
  Demux/3 -> Product5/2
  Pos_ObjectPoint_CoorSys_E[x;y;z][m]/1 -> Demux/1
  Product2/1 -> Mux/1
  Relational Operator1/1 -> Product6/1, Product/1, Product1/1, Product5/1, Product4/1, Product2/1, Product3/1
  Demux/2 -> Product4/2
  Product4/1 -> Mux/2
  Product5/1 -> Mux/3
  Demux/1 -> Product2/2
  Product6/1 -> Object_ID_Masked[]/1

== system ASM_Traffic_MultiCore/Environment/Sensors/UserInterface/DISP_Plant/Object_Sensor_3D/IdxSelect_3DSensor/MaskObjectData_RadarPoints_2 ==
  Object_ID_Expected[] : Inport
  Object_ID[] : Inport  Port=2
  ID[] : Inport  Port=3
  Dist_CoorSys_S[m] : Inport  Port=4
  Angle_Hor_CoorSys_S[deg] : Inport  Port=5
  Pos_ObjectPoint_CoorSys_E[x;y;z][m] : Inport  Port=6
  Demux : Demux  Outputs=3
  Mux : Mux  Inputs=3
  Product{,1..6} (7 alike) : Product
  Relational Operator1 : RelationalOperator  Operator===  OutDataTypeStr=boolean  RndMeth=Simplest  InputSameDT=off
  Object_ID_Masked[] : Outport
  ID_Masked[] : Outport  Port=2
  Dist_CoorSys_S_Masked[m] : Outport  Port=3
  Angle_Hor_CoorSys_S_Masked[deg] : Outport  Port=4
  Pos_ObjectPoint_CoorSys_E_Masked[x;y;z][m] : Outport  Port=5
  wires:
  Dist_CoorSys_S[m]/1 -> Product1/2
  Angle_Hor_CoorSys_S[deg]/1 -> Product3/2
  Mux/1 -> Pos_ObjectPoint_CoorSys_E_Masked[x;y;z][m]/1
  Product/1 -> ID_Masked[]/1
  Object_ID_Expected[]/1 -> Relational Operator1/1
  ID[]/1 -> Product/2
  Product3/1 -> Angle_Hor_CoorSys_S_Masked[deg]/1
  Product1/1 -> Dist_CoorSys_S_Masked[m]/1
  Object_ID[]/1 -> Product6/2, Relational Operator1/2
  Demux/3 -> Product5/2
  Pos_ObjectPoint_CoorSys_E[x;y;z][m]/1 -> Demux/1
  Product2/1 -> Mux/1
  Relational Operator1/1 -> Product6/1, Product/1, Product1/1, Product5/1, Product4/1, Product2/1, Product3/1
  Demux/2 -> Product4/2
  Product4/1 -> Mux/2
  Product5/1 -> Mux/3
  Demux/1 -> Product2/2
  Product6/1 -> Object_ID_Masked[]/1

== system ASM_Traffic_MultiCore/Environment/Sensors/UserInterface/DISP_Plant/Object_Sensor_3D/IdxSelect_3DSensor/MaskObjectData_RadarPoints_3 ==
  Object_ID_Expected[] : Inport
  Object_ID[] : Inport  Port=2
  ID[] : Inport  Port=3
  Dist_CoorSys_S[m] : Inport  Port=4
  Angle_Hor_CoorSys_S[deg] : Inport  Port=5
  Pos_ObjectPoint_CoorSys_E[x;y;z][m] : Inport  Port=6
  Demux : Demux  Outputs=3
  Mux : Mux  Inputs=3
  Product{,1..6} (7 alike) : Product
  Relational Operator1 : RelationalOperator  Operator===  OutDataTypeStr=boolean  RndMeth=Simplest  InputSameDT=off
  Object_ID_Masked[] : Outport
  ID_Masked[] : Outport  Port=2
  Dist_CoorSys_S_Masked[m] : Outport  Port=3
  Angle_Hor_CoorSys_S_Masked[deg] : Outport  Port=4
  Pos_ObjectPoint_CoorSys_E_Masked[x;y;z][m] : Outport  Port=5
  wires:
  Dist_CoorSys_S[m]/1 -> Product1/2
  Angle_Hor_CoorSys_S[deg]/1 -> Product3/2
  Mux/1 -> Pos_ObjectPoint_CoorSys_E_Masked[x;y;z][m]/1
  Product/1 -> ID_Masked[]/1
  Object_ID_Expected[]/1 -> Relational Operator1/1
  ID[]/1 -> Product/2
  Product3/1 -> Angle_Hor_CoorSys_S_Masked[deg]/1
  Product1/1 -> Dist_CoorSys_S_Masked[m]/1
  Object_ID[]/1 -> Product6/2, Relational Operator1/2
  Demux/3 -> Product5/2
  Pos_ObjectPoint_CoorSys_E[x;y;z][m]/1 -> Demux/1
  Product2/1 -> Mux/1
  Relational Operator1/1 -> Product6/1, Product/1, Product1/1, Product5/1, Product4/1, Product2/1, Product3/1
  Demux/2 -> Product4/2
  Product4/1 -> Mux/2
  Product5/1 -> Mux/3
  Demux/1 -> Product2/2
  Product6/1 -> Object_ID_Masked[]/1

== system ASM_Traffic_MultiCore/Environment/Sensors/UserInterface/DISP_Plant/Object_Sensor_3D/IdxSelect_3DSensor/NearestSurf_Index_1[] ==
  In1 : Inport
  Out1 : Outport  VectorParamsAs1DForOutWhenUnconnected=off
  wires:
  In1/1 -> Out1/1

== system ASM_Traffic_MultiCore/Environment/Sensors/UserInterface/DISP_Plant/Object_Sensor_3D/IdxSelect_3DSensor/NearestSurf_Index_2[] ==
  In1 : Inport
  Out1 : Outport  VectorParamsAs1DForOutWhenUnconnected=off
  wires:
  In1/1 -> Out1/1

== system ASM_Traffic_MultiCore/Environment/Sensors/UserInterface/DISP_Plant/Object_Sensor_3D/IdxSelect_3DSensor/NearestSurf_Index_3[] ==
  In1 : Inport
  Out1 : Outport  VectorParamsAs1DForOutWhenUnconnected=off
  wires:
  In1/1 -> Out1/1

== system ASM_Traffic_MultiCore/Environment/Sensors/UserInterface/DISP_Plant/Object_Sensor_3D/IdxSelect_3DSensor/NearestSurf_Pnts_Index_1[] ==
  In1 : Inport
  Out1 : Outport  VectorParamsAs1DForOutWhenUnconnected=off
  wires:
  In1/1 -> Out1/1

== system ASM_Traffic_MultiCore/Environment/Sensors/UserInterface/DISP_Plant/Object_Sensor_3D/IdxSelect_3DSensor/NearestSurf_Pnts_Index_2[] ==
  In1 : Inport
  Out1 : Outport  VectorParamsAs1DForOutWhenUnconnected=off
  wires:
  In1/1 -> Out1/1

== system ASM_Traffic_MultiCore/Environment/Sensors/UserInterface/DISP_Plant/Object_Sensor_3D/IdxSelect_3DSensor/NearestSurf_Pnts_Index_3[] ==
  In1 : Inport
  Out1 : Outport  VectorParamsAs1DForOutWhenUnconnected=off
  wires:
  In1/1 -> Out1/1

== system ASM_Traffic_MultiCore/Environment/Sensors/UserInterface/DISP_Plant/Object_Sensor_3D/IdxSelect_3DSensor/ObjectSample_1[s] ==
  In1 : Inport
  Out1 : Outport  VectorParamsAs1DForOutWhenUnconnected=off
  wires:
  In1/1 -> Out1/1

== system ASM_Traffic_MultiCore/Environment/Sensors/UserInterface/DISP_Plant/Object_Sensor_3D/IdxSelect_3DSensor/ObjectSample_2[s] ==
  In1 : Inport
  Out1 : Outport  VectorParamsAs1DForOutWhenUnconnected=off
  wires:
  In1/1 -> Out1/1

== system ASM_Traffic_MultiCore/Environment/Sensors/UserInterface/DISP_Plant/Object_Sensor_3D/IdxSelect_3DSensor/ObjectSample_3[s] ==
  In1 : Inport
  Out1 : Outport  VectorParamsAs1DForOutWhenUnconnected=off
  wires:
  In1/1 -> Out1/1

== system ASM_Traffic_MultiCore/Environment/Sensors/UserInterface/DISP_Plant/Object_Sensor_3D/IdxSelect_3DSensor/Object_Age_1[s] ==
  In1 : Inport
  Out1 : Outport  VectorParamsAs1DForOutWhenUnconnected=off
  wires:
  In1/1 -> Out1/1

== system ASM_Traffic_MultiCore/Environment/Sensors/UserInterface/DISP_Plant/Object_Sensor_3D/IdxSelect_3DSensor/Object_Age_2[s] ==
  In1 : Inport
  Out1 : Outport  VectorParamsAs1DForOutWhenUnconnected=off
  wires:
  In1/1 -> Out1/1

== system ASM_Traffic_MultiCore/Environment/Sensors/UserInterface/DISP_Plant/Object_Sensor_3D/IdxSelect_3DSensor/Object_Age_3[s] ==
  In1 : Inport
  Out1 : Outport  VectorParamsAs1DForOutWhenUnconnected=off
  wires:
  In1/1 -> Out1/1

== system ASM_Traffic_MultiCore/Environment/Sensors/UserInterface/DISP_Plant/Object_Sensor_3D/IdxSelect_3DSensor/Object_ID_1[] ==
  In1 : Inport
  Out1 : Outport  VectorParamsAs1DForOutWhenUnconnected=off
  wires:
  In1/1 -> Out1/1

== system ASM_Traffic_MultiCore/Environment/Sensors/UserInterface/DISP_Plant/Object_Sensor_3D/IdxSelect_3DSensor/Object_ID_2[] ==
  In1 : Inport
  Out1 : Outport  VectorParamsAs1DForOutWhenUnconnected=off
  wires:
  In1/1 -> Out1/1

== system ASM_Traffic_MultiCore/Environment/Sensors/UserInterface/DISP_Plant/Object_Sensor_3D/IdxSelect_3DSensor/Object_ID_3[] ==
  In1 : Inport
  Out1 : Outport  VectorParamsAs1DForOutWhenUnconnected=off
  wires:
  In1/1 -> Out1/1

== system ASM_Traffic_MultiCore/Environment/Sensors/UserInterface/DISP_Plant/Object_Sensor_3D/IdxSelect_3DSensor/Object_In_Scope_Entry_First_1[s] ==
  In1 : Inport
  Out1 : Outport  VectorParamsAs1DForOutWhenUnconnected=off
  wires:
  In1/1 -> Out1/1

== system ASM_Traffic_MultiCore/Environment/Sensors/UserInterface/DISP_Plant/Object_Sensor_3D/IdxSelect_3DSensor/Object_In_Scope_Entry_First_2[s] ==
  In1 : Inport
  Out1 : Outport  VectorParamsAs1DForOutWhenUnconnected=off
  wires:
  In1/1 -> Out1/1

== system ASM_Traffic_MultiCore/Environment/Sensors/UserInterface/DISP_Plant/Object_Sensor_3D/IdxSelect_3DSensor/Object_In_Scope_Entry_First_3[s] ==
  In1 : Inport
  Out1 : Outport  VectorParamsAs1DForOutWhenUnconnected=off
  wires:
  In1/1 -> Out1/1

== system ASM_Traffic_MultiCore/Environment/Sensors/UserInterface/DISP_Plant/Object_Sensor_3D/IdxSelect_3DSensor/Object_In_Scope_Entry_Number_1[] ==
  In1 : Inport
  Out1 : Outport  VectorParamsAs1DForOutWhenUnconnected=off
  wires:
  In1/1 -> Out1/1

== system ASM_Traffic_MultiCore/Environment/Sensors/UserInterface/DISP_Plant/Object_Sensor_3D/IdxSelect_3DSensor/Object_In_Scope_Entry_Number_2[] ==
  In1 : Inport
  Out1 : Outport  VectorParamsAs1DForOutWhenUnconnected=off
  wires:
  In1/1 -> Out1/1

== system ASM_Traffic_MultiCore/Environment/Sensors/UserInterface/DISP_Plant/Object_Sensor_3D/IdxSelect_3DSensor/Object_In_Scope_Entry_Number_3[] ==
  In1 : Inport
  Out1 : Outport  VectorParamsAs1DForOutWhenUnconnected=off
  wires:
  In1/1 -> Out1/1

== system ASM_Traffic_MultiCore/Environment/Sensors/UserInterface/DISP_Plant/Object_Sensor_3D/IdxSelect_3DSensor/Object_Info_1[-1None|1Fellow|2Static] ==
  In1 : Inport
  Out1 : Outport  VectorParamsAs1DForOutWhenUnconnected=off
  wires:
  In1/1 -> Out1/1

== system ASM_Traffic_MultiCore/Environment/Sensors/UserInterface/DISP_Plant/Object_Sensor_3D/IdxSelect_3DSensor/Object_Info_2[-1None|1Fellow|2Static] ==
  In1 : Inport
  Out1 : Outport  VectorParamsAs1DForOutWhenUnconnected=off
  wires:
  In1/1 -> Out1/1

== system ASM_Traffic_MultiCore/Environment/Sensors/UserInterface/DISP_Plant/Object_Sensor_3D/IdxSelect_3DSensor/Object_Info_3[-1None|1Fellow|2Static] ==
  In1 : Inport
  Out1 : Outport  VectorParamsAs1DForOutWhenUnconnected=off
  wires:
  In1/1 -> Out1/1

== system ASM_Traffic_MultiCore/Environment/Sensors/UserInterface/DISP_Plant/Object_Sensor_3D/IdxSelect_3DSensor/Object_Type_1[] ==
  In1 : Inport
  Out1 : Outport  VectorParamsAs1DForOutWhenUnconnected=off
  wires:
  In1/1 -> Out1/1

== system ASM_Traffic_MultiCore/Environment/Sensors/UserInterface/DISP_Plant/Object_Sensor_3D/IdxSelect_3DSensor/Object_Type_2[] ==
  In1 : Inport
  Out1 : Outport  VectorParamsAs1DForOutWhenUnconnected=off
  wires:
  In1/1 -> Out1/1

== system ASM_Traffic_MultiCore/Environment/Sensors/UserInterface/DISP_Plant/Object_Sensor_3D/IdxSelect_3DSensor/Object_Type_3[] ==
  In1 : Inport
  Out1 : Outport  VectorParamsAs1DForOutWhenUnconnected=off
  wires:
  In1/1 -> Out1/1

== system ASM_Traffic_MultiCore/Environment/Sensors/UserInterface/DISP_Plant/Object_Sensor_3D/IdxSelect_3DSensor/Object_Valid_1[0|1] ==
  In1 : Inport
  Out1 : Outport  VectorParamsAs1DForOutWhenUnconnected=off
  wires:
  In1/1 -> Out1/1

== system ASM_Traffic_MultiCore/Environment/Sensors/UserInterface/DISP_Plant/Object_Sensor_3D/IdxSelect_3DSensor/Object_Valid_2[0|1] ==
  In1 : Inport
  Out1 : Outport  VectorParamsAs1DForOutWhenUnconnected=off
  wires:
  In1/1 -> Out1/1

== system ASM_Traffic_MultiCore/Environment/Sensors/UserInterface/DISP_Plant/Object_Sensor_3D/IdxSelect_3DSensor/Object_Valid_3[0|1] ==
  In1 : Inport
  Out1 : Outport  VectorParamsAs1DForOutWhenUnconnected=off
  wires:
  In1/1 -> Out1/1

== system ASM_Traffic_MultiCore/Environment/Sensors/UserInterface/DISP_Plant/Object_Sensor_3D/IdxSelect_3DSensor/Occlusion_Ratio_Object1[-1|0_1] ==
  In1 : Inport
  Out1 : Outport  VectorParamsAs1DForOutWhenUnconnected=off
  wires:
  In1/1 -> Out1/1

== system ASM_Traffic_MultiCore/Environment/Sensors/UserInterface/DISP_Plant/Object_Sensor_3D/IdxSelect_3DSensor/Occlusion_Ratio_Object2[-1|0_1] ==
  In1 : Inport
  Out1 : Outport  VectorParamsAs1DForOutWhenUnconnected=off
  wires:
  In1/1 -> Out1/1

== system ASM_Traffic_MultiCore/Environment/Sensors/UserInterface/DISP_Plant/Object_Sensor_3D/IdxSelect_3DSensor/Occlusion_Ratio_Object3[-1|0_1] ==
  In1 : Inport
  Out1 : Outport  VectorParamsAs1DForOutWhenUnconnected=off
  wires:
  In1/1 -> Out1/1

== system ASM_Traffic_MultiCore/Environment/Sensors/UserInterface/DISP_Plant/Object_Sensor_3D/IdxSelect_3DSensor/PosVec_x_CenterPnt_Object_1[m] ==
  In1 : Inport
  Out1 : Outport  VectorParamsAs1DForOutWhenUnconnected=off
  wires:
  In1/1 -> Out1/1

== system ASM_Traffic_MultiCore/Environment/Sensors/UserInterface/DISP_Plant/Object_Sensor_3D/IdxSelect_3DSensor/PosVec_x_CenterPnt_Object_2[m] ==
  In1 : Inport
  Out1 : Outport  VectorParamsAs1DForOutWhenUnconnected=off
  wires:
  In1/1 -> Out1/1

== system ASM_Traffic_MultiCore/Environment/Sensors/UserInterface/DISP_Plant/Object_Sensor_3D/IdxSelect_3DSensor/PosVec_x_CenterPnt_Object_3[m] ==
  In1 : Inport
  Out1 : Outport  VectorParamsAs1DForOutWhenUnconnected=off
  wires:
  In1/1 -> Out1/1

== system ASM_Traffic_MultiCore/Environment/Sensors/UserInterface/DISP_Plant/Object_Sensor_3D/IdxSelect_3DSensor/PosVec_y_CenterPnt_Object_1[m] ==
  In1 : Inport
  Out1 : Outport  VectorParamsAs1DForOutWhenUnconnected=off
  wires:
  In1/1 -> Out1/1

== system ASM_Traffic_MultiCore/Environment/Sensors/UserInterface/DISP_Plant/Object_Sensor_3D/IdxSelect_3DSensor/PosVec_y_CenterPnt_Object_2[m] ==
  In1 : Inport
  Out1 : Outport  VectorParamsAs1DForOutWhenUnconnected=off
  wires:
  In1/1 -> Out1/1

== system ASM_Traffic_MultiCore/Environment/Sensors/UserInterface/DISP_Plant/Object_Sensor_3D/IdxSelect_3DSensor/PosVec_y_CenterPnt_Object_3[m] ==
  In1 : Inport
  Out1 : Outport  VectorParamsAs1DForOutWhenUnconnected=off
  wires:
  In1/1 -> Out1/1

== system ASM_Traffic_MultiCore/Environment/Sensors/UserInterface/DISP_Plant/Object_Sensor_3D/IdxSelect_3DSensor/PosVec_z_CenterPnt_Object_1[m] ==
  In1 : Inport
  Out1 : Outport  VectorParamsAs1DForOutWhenUnconnected=off
  wires:
  In1/1 -> Out1/1

== system ASM_Traffic_MultiCore/Environment/Sensors/UserInterface/DISP_Plant/Object_Sensor_3D/IdxSelect_3DSensor/PosVec_z_CenterPnt_Object_2[m] ==
  In1 : Inport
  Out1 : Outport  VectorParamsAs1DForOutWhenUnconnected=off
  wires:
  In1/1 -> Out1/1

== system ASM_Traffic_MultiCore/Environment/Sensors/UserInterface/DISP_Plant/Object_Sensor_3D/IdxSelect_3DSensor/PosVec_z_CenterPnt_Object_3[m] ==
  In1 : Inport
  Out1 : Outport  VectorParamsAs1DForOutWhenUnconnected=off
  wires:
  In1/1 -> Out1/1

== system ASM_Traffic_MultiCore/Environment/Sensors/UserInterface/DISP_Plant/Object_Sensor_3D/IdxSelect_3DSensor/Pos_NearestSurf_Pnt1_CoorSys_S_1[x;y;z][m] ==
  In1 : Inport
  Out1 : Outport  VectorParamsAs1DForOutWhenUnconnected=off
  wires:
  In1/1 -> Out1/1

== system ASM_Traffic_MultiCore/Environment/Sensors/UserInterface/DISP_Plant/Object_Sensor_3D/IdxSelect_3DSensor/Pos_NearestSurf_Pnt1_CoorSys_S_2[x;y;z][m] ==
  In1 : Inport
  Out1 : Outport  VectorParamsAs1DForOutWhenUnconnected=off
  wires:
  In1/1 -> Out1/1

== system ASM_Traffic_MultiCore/Environment/Sensors/UserInterface/DISP_Plant/Object_Sensor_3D/IdxSelect_3DSensor/Pos_NearestSurf_Pnt1_CoorSys_S_3[x;y;z][m] ==
  In1 : Inport
  Out1 : Outport  VectorParamsAs1DForOutWhenUnconnected=off
  wires:
  In1/1 -> Out1/1
